simulink model "OcclusionDetection"  (R2022b)
settings: Solver=FixedStepDiscrete  StartTime=0.0  StopTime=120  MaxStep=0.001  RelTol=1e-5
libraries: dspmtrx3 x3, simulink x1, dspmlti4 x1
settings Model: Creator=szhang  LastModifiedBy=ppatel
settings SolverCC: AlgebraicLoopSolver=TrustRegion
settings DataIOCC: InitialState=simState  LimitDataPoints=on  SaveFinalState=on  SaveOutput=off  SaveTime=off
settings OptimizationCC: DefaultParameterBehavior=Inlined  UseDivisionForNetSlopeComputation=on  UseFloatMulNetSlope=on  InlineInvariantSignals=on  PassReuseOutputArgsAs=Individual arguments  ZeroExternalMemoryAtStartup=off  ZeroInternalMemoryAtStartup=off  NoFixptDivByZeroProtection=on  EfficientFloat2IntCast=on  LifeSpan=Inf  EfficientTunableParamExpr=on
settings DebuggingCC: SignalRangeChecking=error  SolverPrmCheckMsg=warning  IntegerOverflowMsg=error  ParameterTunabilityLossMsg=error  UnconnectedInputMsg=warning  UnconnectedOutputMsg=warning  UnconnectedLineMsg=warning  AssertControl=DisableAll  SFUnexpectedBacktrackingDiag=warning  SFNoUnconditionalDefaultTransitionDiag=warning  SFUnreachableExecutionPathDiag=error  SFExecutionAtInitializationDiag=none  SFMachineParentedDataDiag=warning  ArithmeticOperatorsInVariantConditions=warning
settings HardwareCC: ProdLongLongMode=on
settings ModelReferenceCC: EnableRefExpFcnMdlSchedulingChecks=on  PropagateSignalLabelsOutOfModel=off
settings SFSimCC: SimUseLocalCustomCode=off  MATLABDynamicMemAlloc=off  CustomCodeUndefinedFunction=UseInterfaceOnly
settings RTWCC: Description=Embedded Coder  SystemTargetFile=ert.tlc  GenCodeOnly=on  TemplateMakefile=ert_default_tmf  GenerateReport=on  RTWUseLocalCustomCode=off  IncludeHyperlinkInReport=on  LaunchReport=on  PortableWordSizes=on
settings CodeAppCC: ForceParamTrailComments=on  IgnoreCustomStorageClasses=off  OperatorAnnotations=on  SimulinkDataObjDesc=on  SFDataObjDesc=on  MATLABFcnDesc=on  CustomSymbolStrGlobalVar=rt$N$M  CustomSymbolStrType=$N$M  CustomSymbolStrFcn=$N$M$F  CustomSymbolStrMacro=$N$M  InsertBlockDesc=on  StateflowObjectComments=on  MATLABSourceComments=on  ReqsInCode=on
settings ERTTargetCC: UtilityFuncGeneration=Shared location  MultiwordLength=2048  GenerateSampleERTMain=on  CombineOutputUpdateFcns=off  CombineSignalStateStructs=on  SuppressErrorStatus=on  SupportAbsoluteTime=off  SupportNonFinite=off  SupportComplex=off  ParenthesesLevel=Maximum  CastingMode=Standards  GenerateSharedConstants=off  InlinedParameterPlacement=NonHierarchical  ERTCustomFileTemplate=example_file_process.tlc  ERTFilePackagingFormat=CompactWithDataFile  EnableSignedLeftShifts=off  EnableSignedRightShifts=off
settings ConfigComp: CovEnable=on  CovScope=ReferencedModels  CovIncludeTopModel=off  CovMetricSettings=dcmw  CovHTMLOptions=-sRT=1 -sVT=0 -aTS=1 -bRG=1 -bTC=1 -hTR=0 -nFC=0 -nFD=1 -scm=1 -bcm=1 -xEv=0 -xEM=0  CovSaveCumulativeToWorkspaceVar=on  CovSaveSingleToWorkspaceVar=on  CovCumulativeReport=on  CovModelRefEnable=on  CovExternalEMLEnable=off  CovSFcnEnable=off  DVTestSuiteOptimization=CombinedObjectives (Nonlinear Extended)  DVDetectDeadLogic=on  DVDesignMinMaxCheck=on  DVHarnessSource=Signal Editor  PSResultDir=ps_results_$ModelName$  PSAutoStubLUT=on
settings SimscapeCC: SimscapeNormalizeSystem=off  SimscapeLogType=all  SimscapeLogLimitData=off

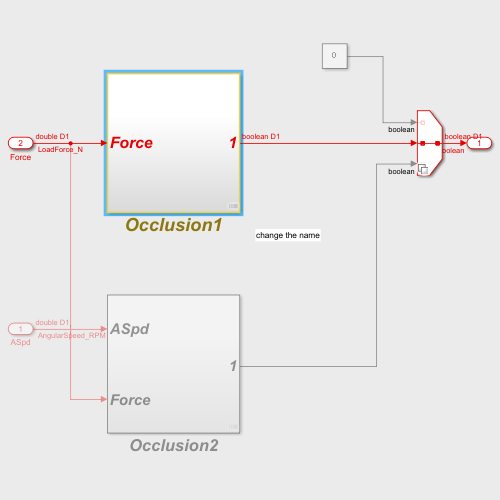
[thumbnail: Simulink's stored preview of the top-level diagram]
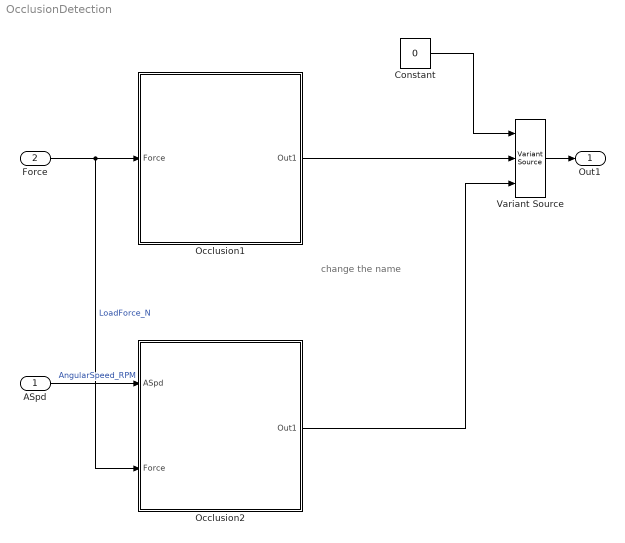
== system OcclusionDetection ==
  note: change the name
  ASpd : Inport  OutDataTypeStr=double  PortDimensions=1  SampleTime=0.001
  Force : Inport  Port=2  OutDataTypeStr=double  PortDimensions=1  SampleTime=0.001
  Constant : Constant  Value=0  OutDataTypeStr=boolean
  Occlusion1 : Subsystem  TreatAsAtomicUnit=on
  Occlusion2 : Subsystem
  Variant Source : VariantSource
  Out1 : Outport  OutDataTypeStr=boolean  PortDimensions=1  SampleTime=0.001  VectorParamsAs1DForOutWhenUnconnected=off
  wires:
  ASpd/1 -> Occlusion2/1(ASpd)  "AngularSpeed_RPM"
  Force/1 -> Occlusion2/2(Force), Occlusion1/1(Force)  "LoadForce_N"
  Occlusion1/1(Out1) -> Variant Source/2
  Variant Source/1 -> Out1/1
  Occlusion2/1(Out1) -> Variant Source/3
  Constant/1 -> Variant Source/1

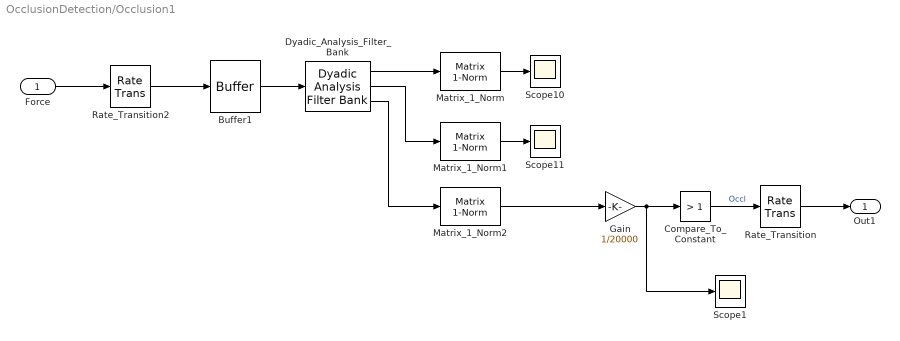
== system OcclusionDetection/Occlusion1 ==
  Force : Inport  OutMin=0  OutMax=10^7
  Buffer1 : Buffer  N=2000  V=1999  OutputFrames=off
  Compare_To_Constant : simulink/Logic and Bit Operations/Compare To Constant  relop=>  const=1  OutDataTypeStr=boolean
  Dyadic_Analysis_Filter_Bank : dspmlti4/Dyadic Analysis Filter Bank  Wname=User-defined  OrdRec_ordDec=[1 / 1]  Order=2  LPF="[0.0352   -0.0854   -0.1350   0.4599   0.8069   0.3327]"  HPF="[-0.3327    0.8069   -0.4599   -0.1350    0.0854    0.0352]"  NumLevels=2  tree=Asymmetric  Output=Multiple ports  OutputFrames=off
  Gain : Gain  Gain=1/20000
  Matrix_1_Norm : dspmtrx3/Matrix  1-Norm  roundingMode=Floor  overflowMode=off  outputDataTypeStr=Inherit: Same as accumulator  outputMin=[]  outputMax=[]  outputLastDataTypeStr=Inherit: Same as accumulator
  Matrix_1_Norm1 : dspmtrx3/Matrix  1-Norm  roundingMode=Floor  overflowMode=off  outputDataTypeStr=Inherit: Same as accumulator  outputMin=[]  outputMax=[]  outputLastDataTypeStr=Inherit: Same as accumulator
  Matrix_1_Norm2 : dspmtrx3/Matrix  1-Norm  roundingMode=Floor  overflowMode=off  outputDataTypeStr=Inherit: Same as accumulator  outputMin=[]  outputMax=[]  outputLastDataTypeStr=Inherit: Same as accumulator
  Rate_Transition : RateTransition
  Rate_Transition2 : RateTransition  OutPortSampleTime=0.01
  Scope1 : Scope
  Scope10 : Scope
  Scope11 : Scope
  Out1 : Outport  OutDataTypeStr=boolean  VectorParamsAs1DForOutWhenUnconnected=off
  wires:
  Rate_Transition/1 -> Out1/1
  Compare_To_Constant/1 -> Rate_Transition/1  "Occl"
  Gain/1 -> Compare_To_Constant/1, Scope1/1
  Matrix_1_Norm2/1 -> Gain/1
  Rate_Transition2/1 -> Buffer1/1
  Force/1 -> Rate_Transition2/1
  Buffer1/1 -> Dyadic_Analysis_Filter_Bank/1
  Matrix_1_Norm/1 -> Scope10/1
  Dyadic_Analysis_Filter_Bank/2 -> Matrix_1_Norm1/1
  Matrix_1_Norm1/1 -> Scope11/1
  Dyadic_Analysis_Filter_Bank/1 -> Matrix_1_Norm/1
  Dyadic_Analysis_Filter_Bank/3 -> Matrix_1_Norm2/1

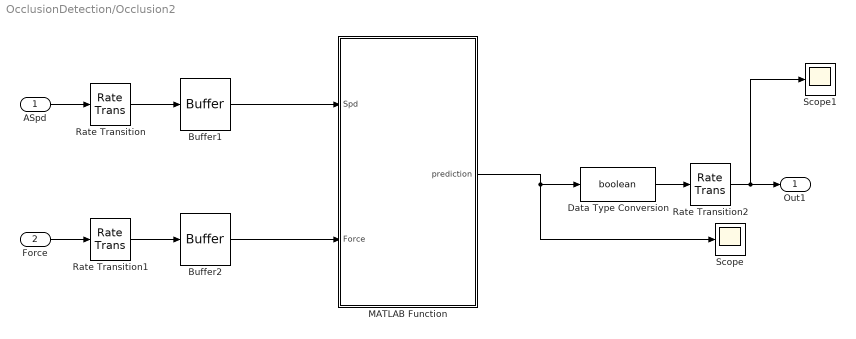
== system OcclusionDetection/Occlusion2 ==
  ASpd : Inport
  Force : Inport  Port=2
  Buffer1 : Buffer  N=2500  OutputFrames=off
  Buffer2 : Buffer  N=2500  OutputFrames=off
  Data Type Conversion : DataTypeConversion  OutDataTypeStr=boolean  SaturateOnIntegerOverflow=off  RndMeth=Floor
  MATLAB Function : MATLAB Function  TreatAsAtomicUnit=on
  Rate Transition : RateTransition  OutPortSampleTime=0.01
  Rate Transition1 : RateTransition  OutPortSampleTime=0.01
  Rate Transition2 : RateTransition  OutPortSampleTime=0.001
  Scope : Scope
  Scope1 : Scope
  Out1 : Outport  VectorParamsAs1DForOutWhenUnconnected=off
  wires:
  MATLAB Function/1(prediction) -> Data Type Conversion/1, Scope/1
  Rate Transition2/1 -> Scope1/1, Out1/1
  Buffer2/1 -> MATLAB Function/2(Force)
  Buffer1/1 -> MATLAB Function/1(Spd)
  Rate Transition1/1 -> Buffer2/1
  Rate Transition/1 -> Buffer1/1
  Force/1 -> Rate Transition1/1
  ASpd/1 -> Rate Transition/1
  Data Type Conversion/1 -> Rate Transition2/1

== matlab function OcclusionDetection/Occlusion2/MATLAB Function ==
  data: Spd input double; prediction output double; Force input double
function prediction = Classification(Spd,Force)
% #codegen
% Define stats function
statfuns = @(x)[max(x) mean(x) min(x) var(x) std(x)];
% Compose all necesssary features
SpdFeature = statfuns(Spd);
ForceFeature = statfuns(Force);
X = [ForceFeature SpdFeature];
% Create  persistent function
persistent CompactMdl

if(isempty(CompactMdl))
    CompactMdl = loadCompactModel('SVMTest3');
end
% Predict classification
prediction = predict(CompactMdl,X);
end
